simulink model "Scissor_Pair_Control_Draft"  (R2025b)
settings: Solver=VariableStepAuto  StartTime=0.0  StopTime=10.0  RelTol=1e-3
values from neighbouring files (symbols this model uses):
  B = 0.005    [Scissor_pair_control_system_script.m]
  J = Izz    (= 3.90625e-05)    [Scissor_pair_control_system_script.m]
  Ke = 1    [Scissor_pair_control_system_script.m]
  Kfoc = 1    [Scissor_pair_control_system_script.m]
  Km = Kt_q/R_ph    [Scissor_pair_control_system_script.m]
undefined symbols (not defined in the file or in its folder): Kv
libraries: cstblocks x2
settings Model: Creator=User  LastModifiedBy=User

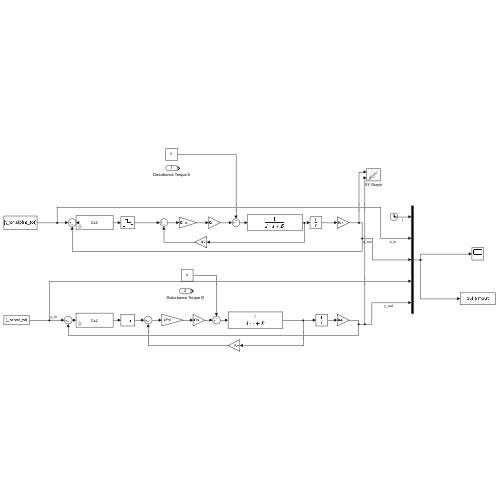
[thumbnail: Simulink's stored preview of the top-level diagram]
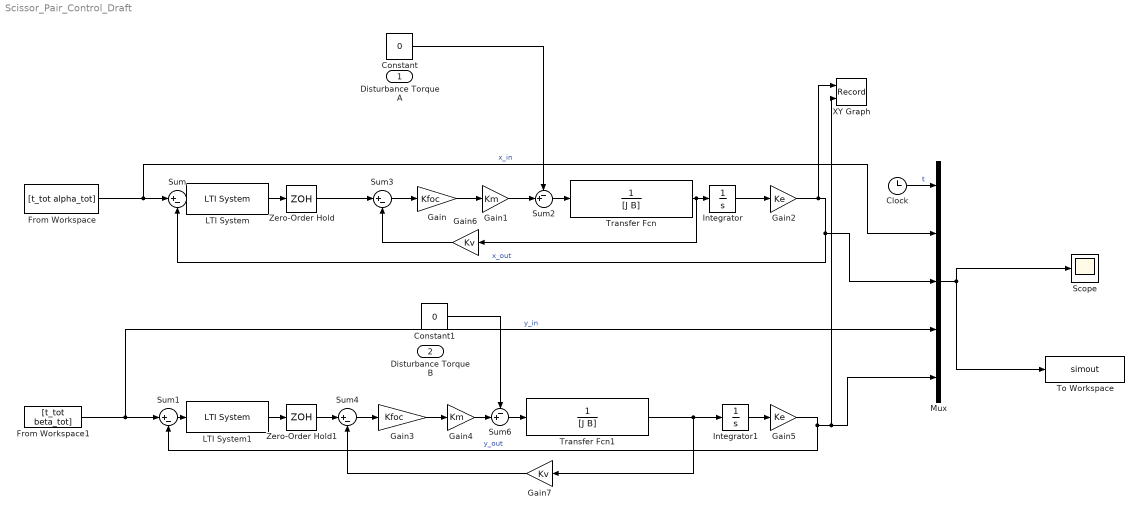
== system Scissor_Pair_Control_Draft ==
  Disturbance Torque A : Inport
  Disturbance Torque B : Inport  Port=2
  Clock : Clock
  Constant : Constant  Value=0
  Constant1 : Constant  Value=0
  From Workspace : FromWorkspace  VariableName=[t_tot alpha_tot]
  From Workspace1 : FromWorkspace  VariableName=[t_tot beta_tot]
  Gain : Gain  Gain=Kfoc
  Gain1 : Gain  Gain=Km
  Gain2 : Gain  Gain=Ke
  Gain3 : Gain  Gain=Kfoc
  Gain4 : Gain  Gain=Km
  Gain5 : Gain  Gain=Ke
  Gain6 : Gain  Gain=Kv
  Gain7 : Gain  Gain=Kv
  Integrator : Integrator
  Integrator1 : Integrator
  LTI System : cstblocks/LTI System  sys=Cz2  IC=[]  PadeOrder=0
  LTI System1 : cstblocks/LTI System  sys=Cz2  IC=[]  PadeOrder=0
  Mux : Mux  Inputs=5
  Scope : Scope
      settings: ActiveDisplayYMinimum=-15.476747744098486  ActiveDisplayYMaximum=135.44321961013313
  Sum{,1,3..4} (4 alike) : Sum  Inputs=|+-
  Sum2 : Sum  Inputs=-+|
  Sum6 : Sum  Inputs=-+|
  To Workspace : ToWorkspace  VariableName=simout  SaveFormat=Timeseries  SampleTime=-1
  Transfer Fcn : TransferFcn  Denominator=[J B]
  Transfer Fcn1 : TransferFcn  Denominator=[J B]
  XY Graph : Record  NumPorts=2.0  FileSettingsInternal="{\"entries\":[{\"content\":{\"excelSettings\":{\"content\":{},\"type\":\"Streamout.ExcelSettings\"},\"parquetSettings\":{\"content\":{},\"type\":\"Streamout.ParquetSettings\"}},\"type\":\"Streamout.FileSettingStorage\",\"uuid\":\"\"}],\"packageUris\":[\"http:\\/\\/schema.mathworks.com\\/mf0\\/streamout_blocks\\/R2020a\"],\"version\":\"1.0\"}"  FrameSettings=[0, 0]  Layout=[1 1]  SignalsInternal="{\"entries\":[{\"content\":{\"signals\":[{\"content\":{\"blockPath\":[],\"dimensions\":[1],\"domain\":\"\",\"lineColor\":\"#a2142f\",\"plots\":[ 1 ],\"port\":1,\"signalID\":1,\"signalName\":\"x_out\"},\"type\":\"RecordBlkView.Signal\",\"uuid\":\"\"},{\"content\":{\"blockPath\":[],\"dimensions\":[1],\"domain\":\"\",\"lineColor\":\"#139fff\",\"plots\":[ 1 ],\"port\":2,\"signalID\":2,\"signalName\":\"y_out\"},\"type\":\"RecordBlkView.Signal\",\"uuid\":\"\"}]},\"type\":\"RecordBlkView.InputSignals\",\"uuid\":\"\"}],\"packageUris\":[\"http:\\/\\/schema.mathworks.com\\/mf0\\/streamout_blocks\\/R2020a\"],\"version\":\"1.0\"}"  VisualizationBindings="{\"xyplotplugin\":{\"info\":[{\"series\":[{\"bindingParametersList\":[{\"parameter\":\"X-Axis\",\"signalID\":1,\"signalName\":\"x_out\"},{\"parameter\":\"Y-Axis\",\"signalID\":2,\"signalName\":\"y_out\"}],\"seriesID\":0}],\"subplotID\":1}]}}"  CompatibilityTag=XY
  Zero-Order Hold : ZeroOrderHold  SampleTime=-1
  Zero-Order Hold1 : ZeroOrderHold  SampleTime=-1
  wires:
  Mux/1 -> To Workspace/1, Scope/1
  Gain3/1 -> Gain4/1
  Sum1/1 -> LTI System1/1
  Clock/1 -> Mux/1  "t"
  From Workspace1/1 -> Sum1/1, Mux/4  "y_in"
  Transfer Fcn/1 -> Gain6/1, Integrator/1
  LTI System/1 -> Zero-Order Hold/1
  Integrator/1 -> Gain2/1
  Gain/1 -> Gain1/1
  Transfer Fcn1/1 -> Gain7/1, Integrator1/1
  Gain5/1 -> XY Graph/2, Mux/5, Sum1/2  "y_out"
  From Workspace/1 -> Sum/1, Mux/2  "x_in"
  Gain2/1 -> XY Graph/1, Sum/2, Mux/3  "x_out"
  Sum/1 -> LTI System/1
  LTI System1/1 -> Zero-Order Hold1/1
  Integrator1/1 -> Gain5/1
  Gain1/1 -> Sum2/2
  Sum2/1 -> Transfer Fcn/1
  Sum6/1 -> Transfer Fcn1/1
  Gain4/1 -> Sum6/2
  Constant/1 -> Sum2/1
  Zero-Order Hold/1 -> Sum3/1
  Sum3/1 -> Gain/1
  Gain6/1 -> Sum3/2
  Zero-Order Hold1/1 -> Sum4/1
  Sum4/1 -> Gain3/1
  Gain7/1 -> Sum4/2
  Constant1/1 -> Sum6/1
